simulink model "FieldControl_PID"  (R2022b)
settings: Solver=VariableStepAuto  StartTime=0.0  StopTime=3  MaxStep=1e-5  RelTol=1e-3
model workspace (MAT data in the model file):
  KI_s = 1
  KP_s = 1
undefined symbols (not defined in the file or in its folder): DiscIntNeverNeededParam
libraries: simulink x2, spspowerguiLib x1
settings Model: SimulationMode=accelerator  Creator=AHMED  LastModifiedBy=moham
settings SolverCC: ZeroCrossAlgorithm=Adaptive
settings DebuggingCC: IgnoredZcDiagnostic=none  UnconnectedInputMsg=warning  UnconnectedOutputMsg=warning  UnconnectedLineMsg=warning
settings ModelReferenceCC: EnableRefExpFcnMdlSchedulingChecks=on
settings RTWCC: DLArmComputeVersion=19.05

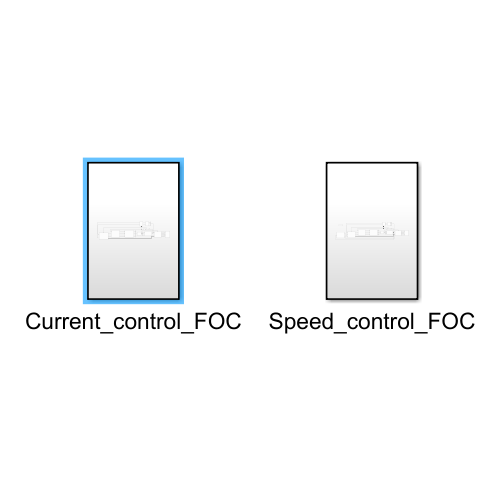
[thumbnail: Simulink's stored preview of the top-level diagram]
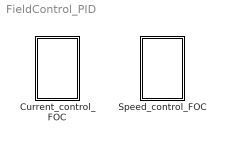
== system FieldControl_PID ==
  Current_control_FOC : Subsystem
  Speed_control_FOC : Subsystem

== system FieldControl_PID/Current_control_FOC ==
  Clark_Transformation : Subsystem
  Control_system : Subsystem
      settings: PortSchema="{\"entries\":[{\"content\":{\"sides\":[{\"content\":{\"connectorIds\":[\"In1\",\"In2\"]},\"type\":\"ConnectorPlacement.EquallySpacedRectSide\",\"uuid\":\"bbdfdf1f-bebb-4c37-9552-0b6c4b897937\"},{\"content\":{\"connectorIds\":[\"Out1\",\"Out2\",\"Out3\"],\"side\":\"RIGHT\"},\"type\":\"ConnectorPlacement.EquallySpacedRectSide\",\"uuid\":\"53bfa961-ba68-4a3a-a1ad-0ed4b4e18017\"},{\"content\":{\"connectorIds\":[\"In3\"],\"side\":\"TOP\"},\"type\":\"ConnectorPlacement.EquallySpacedRectSide\",\"uuid\":\"2095b707-afbd-40f7-b981-0b1948571757\"}]},\"type\":\"ConnectorPlacement.EquallySpacedConnector\",\"uuid\":\"40e57877-c239-4f15-a9c9-ed3794419c45\"}],\"packageUris\":[\"http://schema.mathworks.com/mf0/Connector/R2020b\"],\"version\":\"1.0\"}"
  Demux : Demux  Outputs=3
  Demux1 : Demux  Outputs=3
  Gain : Gain  Gain=2
  Integrator : Integrator
  Inverse_park_clark : Subsystem
  "Inverter " : Subsystem
  Mux : Mux  Inputs=3
  PMSM : Subsystem  mask{Ld=0.0057, Lq=0.0125, lamda_pm=0.123, R=1.2, P=4, J=0.0001, b=0}
  Park_Transformation : Subsystem
      settings: PortSchema="{\"entries\":[{\"content\":{\"sides\":[{\"content\":{\"connectorIds\":[\"In1\",\"In2\"]},\"type\":\"ConnectorPlacement.EquallySpacedRectSide\",\"uuid\":\"a5303260-9056-4ba9-bf21-9d9e68c76aad\"},{\"content\":{\"connectorIds\":[\"Out1\",\"Out2\"],\"side\":\"RIGHT\"},\"type\":\"ConnectorPlacement.EquallySpacedRectSide\",\"uuid\":\"bf8eba39-f781-4672-b99d-9d1cb4b6396f\"},{\"content\":{\"connectorIds\":[],\"side\":\"TOP\"},\"type\":\"ConnectorPlacement.EquallySpacedRectSide\",\"uuid\":\"4985423e-053d-4914-82fe-b9dd9f427f0d\"},{\"content\":{\"connectorIds\":[\"In3\"],\"side\":\"BOTTOM\"},\"type\":\"ConnectorPlacement.EquallySpacedRectSide\",\"uuid\":\"0752c2be-c5bb-44b3-a6b0-4f5b66c2ccb1\"}]},\"type\":\"ConnectorPlacement.EquallySpacedConnector\",\"uuid\":\"0aeb7acd-9c9e-4bf3-9d65-4f157eb3bd0a\"}],\"packageUris\":[\"http://schema.mathworks.com/mf0/Connector/R2020b\"],\"version\":\"1.0\"}"
  SVM : Subsystem
  Scope : Scope  NumInputPorts=8
  Scope_sys : Subsystem
      settings: PortSchema="{\"entries\":[{\"content\":{\"sides\":[{\"content\":{\"connectorIds\":[\"In1\",\"In2\",\"In3\",\"In4\"]},\"type\":\"ConnectorPlacement.EquallySpacedRectSide\",\"uuid\":\"f5ff00d6-72d0-455a-b8b4-a2b5e0f936c9\"},{\"content\":{\"connectorIds\":[\"Out1\",\"Out2\",\"Out3\",\"Out4\",\"Out5\",\"Out6\",\"Out7\",\"Out8\"],\"side\":\"RIGHT\"},\"type\":\"ConnectorPlacement.EquallySpacedRectSide\",\"uuid\":\"90221681-7e43-47d8-9ea8-4435eb27af9a\"},{\"content\":{\"connectorIds\":[\"In5\"],\"side\":\"TOP\"},\"type\":\"ConnectorPlacement.EquallySpacedRectSide\",\"uuid\":\"62fb04f8-341d-442a-bb15-2a5c062453bf\"}]},\"type\":\"ConnectorPlacement.EquallySpacedConnector\",\"uuid\":\"244d1d3d-d937-49d8-9876-c8777bd7e7cc\"}],\"packageUris\":[\"http://schema.mathworks.com/mf0/Connector/R2020b\"],\"version\":\"1.0\"}"
  wires:
  Inverse_park_clark/3(Vc) -> SVM/3(Vc)
  Gain/1 -> Control_system/3(we), Integrator/1
  "Inverter "/1("Voltage ") -> Scope_sys/5("Voltage "), Demux/1
  Inverse_park_clark/2(Vb) -> SVM/2(Vb)
  Demux/3 -> PMSM/3(Vc)
  Clark_Transformation/1(I_alpha) -> Park_Transformation/1(I_alpha)
  SVM/1(S1) -> Mux/1
  Demux/2 -> PMSM/2(Vb)
  SVM/3(S5) -> Mux/3
  Demux1/1 -> Clark_Transformation/1(Ia)
  Clark_Transformation/2(I_beta) -> Park_Transformation/2(I_beta)
  Inverse_park_clark/1(Va) -> SVM/1(Va)
  Mux/1 -> "Inverter "/1("Switches ")
  SVM/2(S3) -> Mux/2
  Control_system/1(Vq) -> Inverse_park_clark/2(Vq)
  Demux1/3 -> Clark_Transformation/3(Ic)
  Integrator/1 -> Park_Transformation/3(theta), Inverse_park_clark/1(theta)
  Control_system/2(Vd) -> Inverse_park_clark/3(Vd)
  Demux1/2 -> Clark_Transformation/2(Ib)
  Demux/1 -> PMSM/1(Va)
  PMSM/1(Stator_currents_Iabc) -> Demux1/1, Scope_sys/1(Iabc)
  PMSM/2(Rotor_speed_Wm) -> Gain/1, Scope_sys/2(Wm)
  PMSM/3(Te) -> Scope_sys/3(Te)
  Park_Transformation/2(I_q) -> Control_system/1(I_q)  "Iq"
  Park_Transformation/1(I_d) -> Control_system/2(I_d)  "Id"
  Control_system/3(Currents) -> Scope_sys/4(Currents)
  Scope_sys/1(Va) -> Scope/1  "Va"
  Scope_sys/2(Vb) -> Scope/2  "Vb"
  Scope_sys/3(Vc) -> Scope/3  "Vc"
  Scope_sys/4(Ia_Ib_Ic) -> Scope/4  "Ia_Ib_Ic"
  Scope_sys/5(Nm) -> Scope/5  "Nm"
  Scope_sys/6(T_ele) -> Scope/6  "Te"
  Scope_sys/7(Iq) -> Scope/7  "Iq"
  Scope_sys/8("Id ") -> Scope/8  "Id"

== system FieldControl_PID/Speed_control_FOC ==
  Clark_Transformation1 : Subsystem
  Current_Control_system : Subsystem
      settings: PortSchema="{\"entries\":[{\"content\":{\"sides\":[{\"content\":{\"connectorIds\":[\"In1\",\"In2\",\"In3\"]},\"type\":\"ConnectorPlacement.EquallySpacedRectSide\",\"uuid\":\"bbdfdf1f-bebb-4c37-9552-0b6c4b897937\"},{\"content\":{\"connectorIds\":[\"Out1\",\"Out2\",\"Out3\"],\"side\":\"RIGHT\"},\"type\":\"ConnectorPlacement.EquallySpacedRectSide\",\"uuid\":\"53bfa961-ba68-4a3a-a1ad-0ed4b4e18017\"},{\"content\":{\"connectorIds\":[\"In4\"],\"side\":\"TOP\"},\"type\":\"ConnectorPlacement.EquallySpacedRectSide\",\"uuid\":\"2095b707-afbd-40f7-b981-0b1948571757\"}]},\"type\":\"ConnectorPlacement.EquallySpacedConnector\",\"uuid\":\"40e57877-c239-4f15-a9c9-ed3794419c45\"}],\"packageUris\":[\"http://schema.mathworks.com/mf0/Connector/R2020b\"],\"version\":\"1.0\"}"
  Demux2 : Demux  Outputs=3
  Demux3 : Demux  Outputs=3
  Gain1 : Gain  Gain=2
  Integrator1 : Integrator
  Inverse_park_clark1 : Subsystem
  Inverter 1 : Subsystem
  Mux1 : Mux  Inputs=3
  PMSM1 : Subsystem  mask{Ld=0.0057, Lq=0.0125, lamda_pm=0.123, R=1.2, P=4, J=0.0001, b=0, TL=4}
  Park_Transformation1 : Subsystem
      settings: PortSchema="{\"entries\":[{\"content\":{\"sides\":[{\"content\":{\"connectorIds\":[\"In1\",\"In2\"]},\"type\":\"ConnectorPlacement.EquallySpacedRectSide\",\"uuid\":\"a5303260-9056-4ba9-bf21-9d9e68c76aad\"},{\"content\":{\"connectorIds\":[\"Out1\",\"Out2\"],\"side\":\"RIGHT\"},\"type\":\"ConnectorPlacement.EquallySpacedRectSide\",\"uuid\":\"bf8eba39-f781-4672-b99d-9d1cb4b6396f\"},{\"content\":{\"connectorIds\":[],\"side\":\"TOP\"},\"type\":\"ConnectorPlacement.EquallySpacedRectSide\",\"uuid\":\"4985423e-053d-4914-82fe-b9dd9f427f0d\"},{\"content\":{\"connectorIds\":[\"In3\"],\"side\":\"BOTTOM\"},\"type\":\"ConnectorPlacement.EquallySpacedRectSide\",\"uuid\":\"0752c2be-c5bb-44b3-a6b0-4f5b66c2ccb1\"}]},\"type\":\"ConnectorPlacement.EquallySpacedConnector\",\"uuid\":\"0aeb7acd-9c9e-4bf3-9d65-4f157eb3bd0a\"}],\"packageUris\":[\"http://schema.mathworks.com/mf0/Connector/R2020b\"],\"version\":\"1.0\"}"
  SVM : Subsystem
  Scope3 : Scope  NumInputPorts=8
  Scope_sys : Subsystem
      settings: PortSchema="{\"entries\":[{\"content\":{\"sides\":[{\"content\":{\"connectorIds\":[\"In1\",\"In2\",\"In3\",\"In4\",\"In5\"]},\"type\":\"ConnectorPlacement.EquallySpacedRectSide\",\"uuid\":\"f5ff00d6-72d0-455a-b8b4-a2b5e0f936c9\"},{\"content\":{\"connectorIds\":[\"Out1\",\"Out2\",\"Out3\",\"Out4\",\"Out5\",\"Out6\",\"Out7\",\"Out8\"],\"side\":\"RIGHT\"},\"type\":\"ConnectorPlacement.EquallySpacedRectSide\",\"uuid\":\"90221681-7e43-47d8-9ea8-4435eb27af9a\"},{\"content\":{\"connectorIds\":[\"In6\"],\"side\":\"TOP\"},\"type\":\"ConnectorPlacement.EquallySpacedRectSide\",\"uuid\":\"62fb04f8-341d-442a-bb15-2a5c062453bf\"}]},\"type\":\"ConnectorPlacement.EquallySpacedConnector\",\"uuid\":\"244d1d3d-d937-49d8-9876-c8777bd7e7cc\"}],\"packageUris\":[\"http://schema.mathworks.com/mf0/Connector/R2020b\"],\"version\":\"1.0\"}"
  Speed_Control_system : Subsystem
  powergui : spspowerguiLib/powergui  Priority=1  SimulationMode=Continuous  SampleTime=50e-6  frequency=60  Iterations=50  frequencyindice=0  Pbase=100e6  ErrMax=1e-4  UnitsV=kV  UnitsW=MW  buscounter=0  FunctionMessages=off  echomessages=off  EnableUseOfTLC=off  CurrentSourceSwitches=off  DisableSnubberDevices=off  DisableRonSwitches=off  DisableVfSwitches=off  DisplayEquations=off  AutomaticDiscreteSolvers=off  SolverType=Tustin/Backward Euler (TBE)  Interpol=off  ExternalGateDelay=off  methode=off  Ts=100  x0status=blocks  SPID=on  SwTol=0  HookPort=off  NonlinearTolerance=1e-4  nMaxIteration=100  ContinueOnMaxIteration=off  RestoreLinks=warning  ResistiveCurrentMeasurement=off  Frange=[0:2:500]  Ylog=off  Xlog=on  ShowGrid=off  save=off  variable=ZData  structure=0  ZoomFFT=off  StartTime=0.0  cycles=1  DisplayStyle=1  fundamental=60  FreqAxis=off  MaxFrequency=1000  frequencyindicesteady=1  RmsSteady=1  display=off
  wires:
  Current_Control_system/3(Currents) -> Scope_sys/4(Currents)
  Scope_sys/8("Id ") -> Scope3/8  "Id"
  PMSM1/3(Te) -> Scope_sys/3(Te)
  Scope_sys/2(Vb) -> Scope3/2  "Vb"
  Demux3/3 -> Clark_Transformation1/3(Ic)
  Scope_sys/6(T_ele) -> Scope3/6  "Te"
  Scope_sys/3(Vc) -> Scope3/3  "Vc"
  PMSM1/1(Stator_currents_Iabc) -> Demux3/1, Scope_sys/1(Iabc)
  Scope_sys/1(Va) -> Scope3/1  "Va"
  PMSM1/2(Rotor_speed_Wm) -> Gain1/1, Scope_sys/2(Wm), Speed_Control_system/1(Wm)
  Scope_sys/7(Iq) -> Scope3/7  "Iq"
  Scope_sys/4(Ia_Ib_Ic) -> Scope3/4  "Ia_Ib_Ic"
  Mux1/1 -> Inverter 1/1("Switches ")
  Park_Transformation1/2(I_q) -> Current_Control_system/1(I_q)  "Iq"
  Scope_sys/5(Nm) -> Scope3/5  "Nm"
  Demux2/1 -> PMSM1/1(Va)
  Demux2/3 -> PMSM1/3(Vc)
  Demux3/2 -> Clark_Transformation1/2(Ib)
  Integrator1/1 -> Park_Transformation1/3(theta), Inverse_park_clark1/1(theta)
  Current_Control_system/2(Vd) -> Inverse_park_clark1/3(Vd)
  Clark_Transformation1/2(I_beta) -> Park_Transformation1/2(I_beta)
  Clark_Transformation1/1(I_alpha) -> Park_Transformation1/1(I_alpha)
  Inverter 1/1("Voltage ") -> Scope_sys/6("Voltage "), Demux2/1
  Park_Transformation1/1(I_d) -> Current_Control_system/2(I_d)  "Id"
  SVM/1(S1) -> Mux1/1
  Inverse_park_clark1/2(Vb) -> SVM/2(Vb)
  Inverse_park_clark1/1(Va) -> SVM/1(Va)
  Current_Control_system/1(Vq) -> Inverse_park_clark1/2(Vq)
  SVM/2(S2) -> Mux1/2
  Demux2/2 -> PMSM1/2(Vb)
  SVM/3(S3) -> Mux1/3
  Demux3/1 -> Clark_Transformation1/1(Ia)
  Inverse_park_clark1/3(Vc) -> SVM/3(Vc)
  Gain1/1 -> Current_Control_system/4(we), Integrator1/1
  Speed_Control_system/1(Iq_ref) -> Current_Control_system/3(Iq_ref)
  Speed_Control_system/2(Wm_ref) -> Scope_sys/5(Wm_ref)

== system FieldControl_PID/Current_control_FOC/Clark_Transformation ==
  Ia : Inport
  Ib : Inport  Port=2
  Ic : Inport  Port=3
  Add : Sum  Inputs=+++
  Add1 : Sum
  Gain : Gain  Gain=-0.5
  Gain1 : Gain  Gain=-0.5
  Gain2 : Gain  Gain=2/3
  Gain3 : Gain  Gain=sqrt(3)/2
  Gain4 : Gain  Gain=-sqrt(3)/2
  Gain5 : Gain  Gain=2/3
  I_alpha : Outport
  I_beta : Outport  Port=2
  wires:
  Ib/1 -> Gain3/1, Gain/1
  Ic/1 -> Gain4/1, Gain1/1
  Gain/1 -> Add/2
  Gain1/1 -> Add/3
  Ia/1 -> Add/1
  Add/1 -> Gain2/1
  Gain2/1 -> I_alpha/1
  Gain4/1 -> Add1/2
  Gain3/1 -> Add1/1
  Add1/1 -> Gain5/1
  Gain5/1 -> I_beta/1

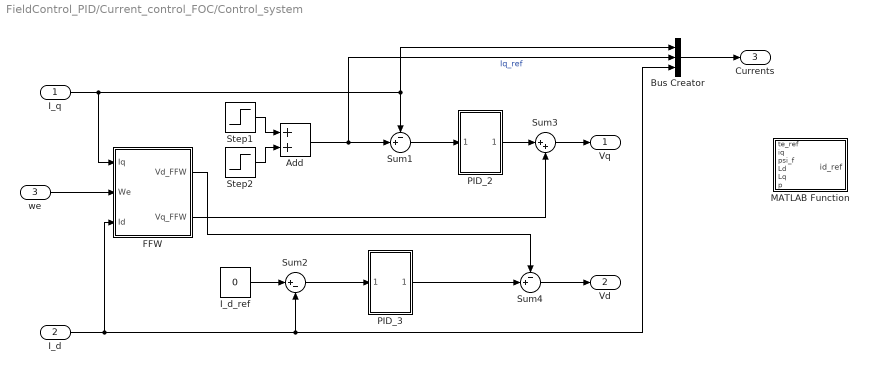
== system FieldControl_PID/Current_control_FOC/Control_system ==
  I_q : Inport
  I_d : Inport  Port=2
  we : Inport  Port=3
  Add : Sum
  Bus Creator : BusCreator  Inputs=3
  FFW : Subsystem
  I_d_ref : Constant  Value=0
  MATLAB Function : MATLAB Function  TreatAsAtomicUnit=on
  PID_2 : Subsystem
  PID_3 : Subsystem
  Step1 : Step  Before=5  After=10  SampleTime=0
  Step2 : Step  Time=2  After=5  SampleTime=0
  Sum1 : Sum  Inputs=-+|
  Sum2 : Sum  Inputs=|+-
  Sum3 : Sum  Inputs=|++
  Sum4 : Sum  Inputs=-+|
  Vq : Outport
  Vd : Outport  Port=2
  Currents : Outport  Port=3
  wires:
  I_q/1 -> FFW/1(Iq), Bus Creator/1, Sum1/1
  Sum1/1 -> PID_2/1(In1)
  I_d/1 -> FFW/3(Id), Bus Creator/3, Sum2/2
  I_d_ref/1 -> Sum2/1
  Sum2/1 -> PID_3/1(In1)
  Add/1 -> Bus Creator/2, Sum1/2  "Iq_ref"
  Bus Creator/1 -> Currents/1
  Sum3/1 -> Vq/1
  PID_3/1(Out1) -> Sum4/2
  Sum4/1 -> Vd/1
  PID_2/1(Out1) -> Sum3/1
  we/1 -> FFW/2(We)
  Step1/1 -> Add/1
  Step2/1 -> Add/2
  FFW/2(Vq_FFW) -> Sum3/2
  FFW/1(Vd_FFW) -> Sum4/1

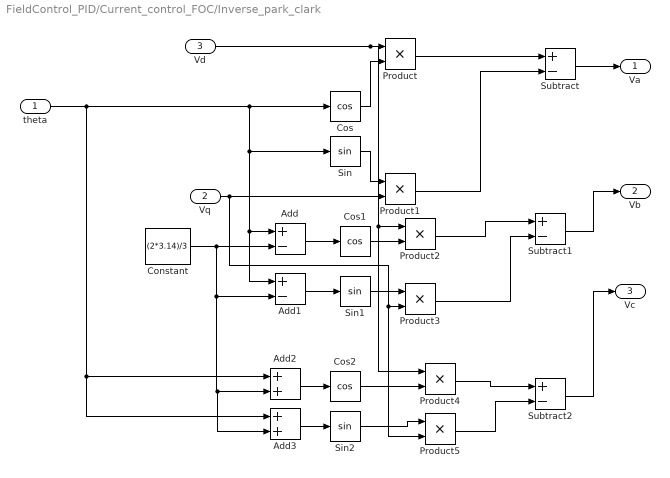
== system FieldControl_PID/Current_control_FOC/Inverse_park_clark ==
  theta : Inport
  Vq : Inport  Port=2
  Vd : Inport  Port=3
  Add : Sum  Inputs=+-
  Add1 : Sum  Inputs=+-
  Add2 : Sum
  Add3 : Sum
  Constant : Constant  Value=(2*3.14)/3
  Cos : Trigonometry  Operator=cos
  Cos1 : Trigonometry  Operator=cos
  Cos2 : Trigonometry  Operator=cos
  Product{,1..5} (6 alike) : Product
  Sin : Trigonometry
  Sin1 : Trigonometry
  Sin2 : Trigonometry
  Subtract : Sum  Inputs=+-
  Subtract1 : Sum  Inputs=+-
  Subtract2 : Sum  Inputs=+-
  Va : Outport
  Vb : Outport  Port=2
  Vc : Outport  Port=3
  wires:
  Subtract/1 -> Va/1
  theta/1 -> Add3/1, Add2/1, Cos/1, Add1/1, Add/1, Sin/1
  Vd/1 -> Product4/1, Product2/1, Product/1
  Cos/1 -> Product/2
  Product/1 -> Subtract/1
  Vq/1 -> Product5/2, Product3/2, Product1/2
  Sin/1 -> Product1/1
  Product1/1 -> Subtract/2
  Add/1 -> Cos1/1
  Add1/1 -> Sin1/1
  Cos1/1 -> Product2/2
  Sin1/1 -> Product3/1
  Product2/1 -> Subtract1/1
  Product3/1 -> Subtract1/2
  Subtract1/1 -> Vb/1
  Constant/1 -> Add3/2, Add2/2, Add1/2, Add/2
  Subtract2/1 -> Vc/1
  Product4/1 -> Subtract2/1
  Product5/1 -> Subtract2/2
  Cos2/1 -> Product4/2
  Sin2/1 -> Product5/1
  Add2/1 -> Cos2/1
  Add3/1 -> Sin2/1

== system FieldControl_PID/Current_control_FOC/Inverter  ==
  "Switches " : Inport
  Fcn : Fcn  Expr=540/3*(2*u(1)-u(2)-u(3))
  Fcn1 : Fcn  Expr=540/3*(2*u(2)-u(1)-u(3))
  Fcn2 : Fcn  Expr=540/3*(2*u(3)-u(2)-u(1))
  Mux1 : Mux  Inputs=3
  "Voltage " : Outport  VectorParamsAs1DForOutWhenUnconnected=off
  wires:
  Mux1/1 -> "Voltage "/1
  Fcn1/1 -> Mux1/2
  "Switches "/1 -> Fcn2/1, Fcn1/1, Fcn/1
  Fcn/1 -> Mux1/1
  Fcn2/1 -> Mux1/3

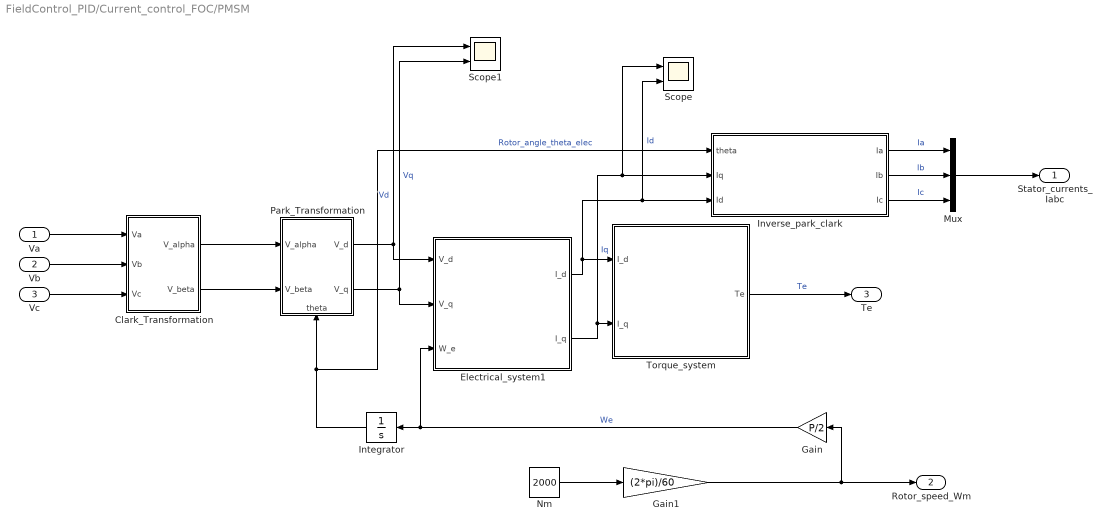
== system FieldControl_PID/Current_control_FOC/PMSM ==
  Va : Inport
  Vb : Inport  Port=2
  Vc : Inport  Port=3
  Clark_Transformation : Subsystem
  Electrical_system1 : Subsystem
  Gain : Gain  Gain=P/2
  Gain1 : Gain  Gain=(2*pi)/60
  Integrator : Integrator
  Inverse_park_clark : Subsystem
  Mux : Mux  Inputs=3
  Nm : Constant  Value=2000
  Park_Transformation : Subsystem
      settings: PortSchema="{\"entries\":[{\"content\":{\"sides\":[{\"content\":{\"connectorIds\":[\"In1\",\"In2\"]},\"type\":\"ConnectorPlacement.EquallySpacedRectSide\",\"uuid\":\"a5303260-9056-4ba9-bf21-9d9e68c76aad\"},{\"content\":{\"connectorIds\":[\"Out1\",\"Out2\"],\"side\":\"RIGHT\"},\"type\":\"ConnectorPlacement.EquallySpacedRectSide\",\"uuid\":\"bf8eba39-f781-4672-b99d-9d1cb4b6396f\"},{\"content\":{\"connectorIds\":[],\"side\":\"TOP\"},\"type\":\"ConnectorPlacement.EquallySpacedRectSide\",\"uuid\":\"4985423e-053d-4914-82fe-b9dd9f427f0d\"},{\"content\":{\"connectorIds\":[\"In3\"],\"side\":\"BOTTOM\"},\"type\":\"ConnectorPlacement.EquallySpacedRectSide\",\"uuid\":\"0752c2be-c5bb-44b3-a6b0-4f5b66c2ccb1\"}]},\"type\":\"ConnectorPlacement.EquallySpacedConnector\",\"uuid\":\"0aeb7acd-9c9e-4bf3-9d65-4f157eb3bd0a\"}],\"packageUris\":[\"http://schema.mathworks.com/mf0/Connector/R2020b\"],\"version\":\"1.0\"}"
  Scope : Scope  NumInputPorts=2
  Scope1 : Scope  NumInputPorts=2
  Torque_system : Subsystem
  Stator_currents_Iabc : Outport
  Rotor_speed_Wm : Outport  Port=2
  Te : Outport  Port=3
  wires:
  Va/1 -> Clark_Transformation/1(Va)
  Vb/1 -> Clark_Transformation/2(Vb)
  Vc/1 -> Clark_Transformation/3(Vc)
  Clark_Transformation/1(V_alpha) -> Park_Transformation/1(V_alpha)
  Clark_Transformation/2(V_beta) -> Park_Transformation/2(V_beta)
  Park_Transformation/1(V_d) -> Electrical_system1/1(V_d), Scope1/1  "Vd"
  Park_Transformation/2(V_q) -> Electrical_system1/2(V_q), Scope1/2  "Vq"
  Electrical_system1/1(I_d) -> Torque_system/1(I_d), Scope/2, Inverse_park_clark/3(Id)  "Id"
  Electrical_system1/2(I_q) -> Scope/1, Inverse_park_clark/2(Iq), Torque_system/2(I_q)  "Iq"
  Torque_system/1(Te) -> Te/1  "Te"
  Gain/1 -> Electrical_system1/3(W_e), Integrator/1  "We"
  Integrator/1 -> Inverse_park_clark/1(theta), Park_Transformation/3(theta)  "Rotor_angle_theta_elec"
  Inverse_park_clark/1(Ia) -> Mux/1  "Ia"
  Inverse_park_clark/2(Ib) -> Mux/2  "Ib"
  Inverse_park_clark/3(Ic) -> Mux/3  "Ic"
  Mux/1 -> Stator_currents_Iabc/1
  Nm/1 -> Gain1/1
  Gain1/1 -> Rotor_speed_Wm/1, Gain/1

== system FieldControl_PID/Current_control_FOC/Park_Transformation ==
  I_alpha : Inport
  I_beta : Inport  Port=2
  theta : Inport  Port=3
  Add : Sum
  Add1 : Sum
  Cos : Trigonometry  Operator=cos
  Cos1 : Trigonometry
  Gain : Gain  Gain=-1
  Product{,1..3} (4 alike) : Product
  I_d : Outport
  I_q : Outport  Port=2
  wires:
  theta/1 -> Cos1/1, Cos/1
  I_alpha/1 -> Product2/1, Product/1
  Cos/1 -> Product3/2, Product/2
  Cos1/1 -> Product2/2, Product1/1
  I_beta/1 -> Product3/1, Product1/2
  Product/1 -> Add/1
  Product1/1 -> Add/2
  Add/1 -> I_d/1
  Product2/1 -> Gain/1
  Gain/1 -> Add1/1
  Product3/1 -> Add1/2
  Add1/1 -> I_q/1

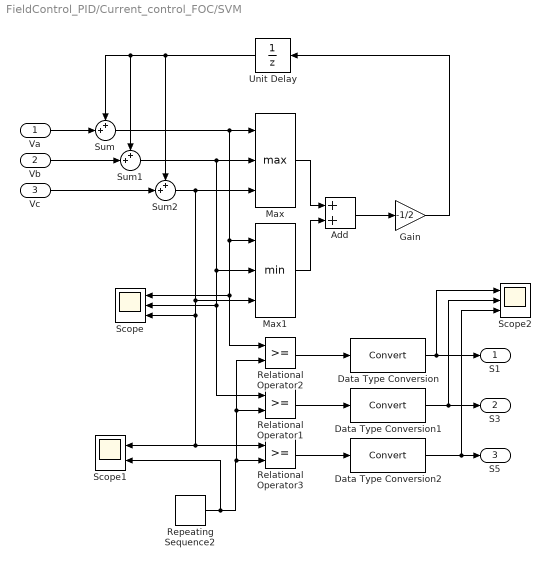
== system FieldControl_PID/Current_control_FOC/SVM ==
  Va : Inport
  Vb : Inport  Port=2
  Vc : Inport  Port=3
  Add : Sum
  Data Type Conversion : DataTypeConversion  SaturateOnIntegerOverflow=off  RndMeth=Floor
  Data Type Conversion1 : DataTypeConversion  SaturateOnIntegerOverflow=off  RndMeth=Floor
  Data Type Conversion2 : DataTypeConversion  SaturateOnIntegerOverflow=off  RndMeth=Floor
  Gain : Gain  Gain=-1/2
  Max : MinMax  Function=max  Inputs=3
  Max1 : MinMax  Inputs=3
  Relational Operator1 : RelationalOperator  OutDataTypeStr=boolean  RndMeth=Simplest  InputSameDT=off
  Relational Operator2 : RelationalOperator  OutDataTypeStr=boolean  RndMeth=Simplest  InputSameDT=off
  Relational Operator3 : RelationalOperator  OutDataTypeStr=boolean  RndMeth=Simplest  InputSameDT=off
  Repeating Sequence2 : simulink/Sources/Repeating Sequence  rep_seq_t=[0 0.5/10000 1/10000]  rep_seq_y=[-280 280 -280]
  Scope : Scope  NumInputPorts=3
  Scope1 : Scope  NumInputPorts=2
  Scope2 : Scope  NumInputPorts=3
  Sum : Sum  Inputs=++|
  Sum1 : Sum  Inputs=++|
  Sum2 : Sum  Inputs=++|
  Unit Delay : UnitDelay  SampleTime=-1  HasFrameUpgradeWarning=on
  S1 : Outport
  S3 : Outport  Port=2
  S5 : Outport  Port=3
  wires:
  Max/1 -> Add/1
  Max1/1 -> Add/2
  Add/1 -> Gain/1
  Data Type Conversion/1 -> Scope2/1, S1/1
  Data Type Conversion1/1 -> Scope2/2, S3/1
  Data Type Conversion2/1 -> Scope2/3, S5/1
  Gain/1 -> Unit Delay/1
  Unit Delay/1 -> Sum1/1, Sum/1, Sum2/1
  Va/1 -> Sum/2
  Vb/1 -> Sum1/2
  Vc/1 -> Sum2/2
  Sum/1 -> Scope/1, Relational Operator2/1, Max1/1, Max/1
  Sum1/1 -> Scope/2, Relational Operator1/1, Max1/2, Max/2
  Sum2/1 -> Scope/3, Scope1/1, Relational Operator3/1, Max1/3, Max/3
  Repeating Sequence2/1 -> Scope1/2, Relational Operator2/2, Relational Operator1/2, Relational Operator3/2
  Relational Operator2/1 -> Data Type Conversion/1
  Relational Operator1/1 -> Data Type Conversion1/1
  Relational Operator3/1 -> Data Type Conversion2/1

== system FieldControl_PID/Current_control_FOC/Scope_sys ==
  Iabc : Inport
  Wm : Inport  Port=2
  Te : Inport  Port=3
  Currents : Inport  Port=4
  "Voltage " : Inport  Port=5
  Bus Selector : BusSelector  OutputSignals=Iq,Iq_ref,Id
  Demux : Demux  Outputs=3
  Gain : Gain  Gain=60/(2*pi)
  Mux : Mux  Inputs=2
  Va : Outport
  Vb : Outport  Port=2
  Vc : Outport  Port=3
  Ia_Ib_Ic : Outport  Port=4
  Nm : Outport  Port=5
  T_ele : Outport  Port=6
  Iq : Outport  Port=7
  "Id " : Outport  Port=8
  wires:
  "Voltage "/1 -> Demux/1
  Demux/1 -> Va/1
  Demux/2 -> Vb/1
  Demux/3 -> Vc/1
  Iabc/1 -> Ia_Ib_Ic/1
  Wm/1 -> Gain/1
  Gain/1 -> Nm/1
  Te/1 -> T_ele/1
  Currents/1 -> Bus Selector/1
  Bus Selector/1 -> Mux/1  "<Iq>"
  Bus Selector/2 -> Mux/2  "<Iq_ref>"
  Bus Selector/3 -> "Id "/1  "<Id>"
  Mux/1 -> Iq/1

== system FieldControl_PID/Speed_control_FOC/Clark_Transformation1 ==
  Ia : Inport
  Ib : Inport  Port=2
  Ic : Inport  Port=3
  Add : Sum  Inputs=+++
  Add1 : Sum
  Gain : Gain  Gain=-0.5
  Gain1 : Gain  Gain=-0.5
  Gain2 : Gain  Gain=2/3
  Gain3 : Gain  Gain=sqrt(3)/2
  Gain4 : Gain  Gain=-sqrt(3)/2
  Gain5 : Gain  Gain=2/3
  I_alpha : Outport
  I_beta : Outport  Port=2
  wires:
  Ib/1 -> Gain3/1, Gain/1
  Ic/1 -> Gain4/1, Gain1/1
  Gain/1 -> Add/2
  Gain1/1 -> Add/3
  Ia/1 -> Add/1
  Add/1 -> Gain2/1
  Gain2/1 -> I_alpha/1
  Gain4/1 -> Add1/2
  Gain3/1 -> Add1/1
  Add1/1 -> Gain5/1
  Gain5/1 -> I_beta/1

== system FieldControl_PID/Speed_control_FOC/Current_Control_system ==
  I_q : Inport
  I_d : Inport  Port=2
  Iq_ref : Inport  Port=3
  we : Inport  Port=4
  Bus Creator : BusCreator  Inputs=3
  I_d_ref : Constant  Value=0
  PID_2 : Subsystem
  PID_3 : Subsystem
  Subsystem : Subsystem
  Sum1 : Sum  Inputs=-+|
  Sum2 : Sum  Inputs=|+-
  Sum3 : Sum  Inputs=|++
  Sum4 : Sum  Inputs=-+|
  Vq : Outport
  Vd : Outport  Port=2
  Currents : Outport  Port=3
  wires:
  I_q/1 -> Subsystem/1(Iq), Bus Creator/1, Sum1/1
  Sum1/1 -> PID_2/1(In1)
  I_d/1 -> Subsystem/3(Id), Bus Creator/3, Sum2/2
  Sum2/1 -> PID_3/1(In1)
  Iq_ref/1 -> Bus Creator/2, Sum1/2  "Iq_ref"
  Bus Creator/1 -> Currents/1
  Sum3/1 -> Vq/1
  PID_3/1(Out1) -> Sum4/2
  Sum4/1 -> Vd/1
  PID_2/1(Out1) -> Sum3/1
  we/1 -> Subsystem/2(We)
  Subsystem/1(Vd_FFW) -> Sum4/1
  Subsystem/2(Vq_FFW) -> Sum3/2
  I_d_ref/1 -> Sum2/1

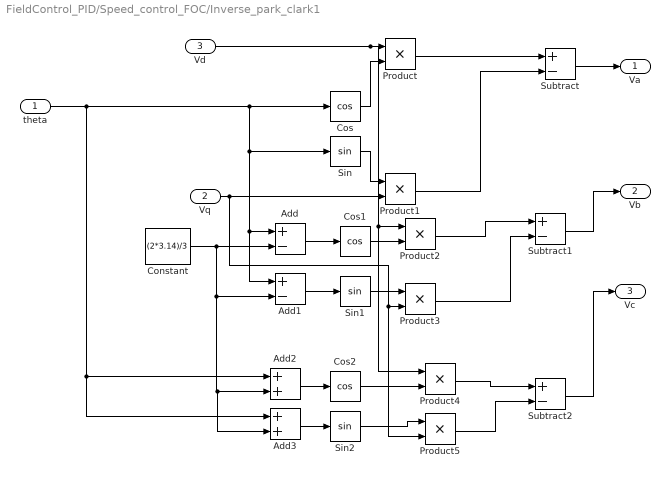
== system FieldControl_PID/Speed_control_FOC/Inverse_park_clark1 ==
  theta : Inport
  Vq : Inport  Port=2
  Vd : Inport  Port=3
  Add : Sum  Inputs=+-
  Add1 : Sum  Inputs=+-
  Add2 : Sum
  Add3 : Sum
  Constant : Constant  Value=(2*3.14)/3
  Cos : Trigonometry  Operator=cos
  Cos1 : Trigonometry  Operator=cos
  Cos2 : Trigonometry  Operator=cos
  Product{,1..5} (6 alike) : Product
  Sin : Trigonometry
  Sin1 : Trigonometry
  Sin2 : Trigonometry
  Subtract : Sum  Inputs=+-
  Subtract1 : Sum  Inputs=+-
  Subtract2 : Sum  Inputs=+-
  Va : Outport
  Vb : Outport  Port=2
  Vc : Outport  Port=3
  wires:
  Subtract/1 -> Va/1
  theta/1 -> Add3/1, Add2/1, Cos/1, Add1/1, Add/1, Sin/1
  Vd/1 -> Product4/1, Product2/1, Product/1
  Cos/1 -> Product/2
  Product/1 -> Subtract/1
  Vq/1 -> Product5/2, Product3/2, Product1/2
  Sin/1 -> Product1/1
  Product1/1 -> Subtract/2
  Add/1 -> Cos1/1
  Add1/1 -> Sin1/1
  Cos1/1 -> Product2/2
  Sin1/1 -> Product3/1
  Product2/1 -> Subtract1/1
  Product3/1 -> Subtract1/2
  Subtract1/1 -> Vb/1
  Constant/1 -> Add3/2, Add2/2, Add1/2, Add/2
  Subtract2/1 -> Vc/1
  Product4/1 -> Subtract2/1
  Product5/1 -> Subtract2/2
  Cos2/1 -> Product4/2
  Sin2/1 -> Product5/1
  Add2/1 -> Cos2/1
  Add3/1 -> Sin2/1

== system FieldControl_PID/Speed_control_FOC/Inverter 1 ==
  "Switches " : Inport
  Fcn : Fcn  Expr=540/3*(2*u(1)-u(2)-u(3))
  Fcn1 : Fcn  Expr=540/3*(2*u(2)-u(1)-u(3))
  Fcn2 : Fcn  Expr=540/3*(2*u(3)-u(2)-u(1))
  Mux1 : Mux  Inputs=3
  "Voltage " : Outport  VectorParamsAs1DForOutWhenUnconnected=off
  wires:
  Mux1/1 -> "Voltage "/1
  Fcn1/1 -> Mux1/2
  "Switches "/1 -> Fcn2/1, Fcn1/1, Fcn/1
  Fcn/1 -> Mux1/1
  Fcn2/1 -> Mux1/3

== system FieldControl_PID/Speed_control_FOC/PMSM1 ==
  Va : Inport
  Vb : Inport  Port=2
  Vc : Inport  Port=3
  Clark_Transformation : Subsystem
  Electrical_system2 : Subsystem
  Gain : Gain  Gain=P/2
  Integrator : Integrator
  Inverse_park_clark : Subsystem
  Mechanical_system : Subsystem
  Mux : Mux  Inputs=3
  Park_Transformation : Subsystem
      settings: PortSchema="{\"entries\":[{\"content\":{\"sides\":[{\"content\":{\"connectorIds\":[\"In1\",\"In2\"]},\"type\":\"ConnectorPlacement.EquallySpacedRectSide\",\"uuid\":\"a5303260-9056-4ba9-bf21-9d9e68c76aad\"},{\"content\":{\"connectorIds\":[\"Out1\",\"Out2\"],\"side\":\"RIGHT\"},\"type\":\"ConnectorPlacement.EquallySpacedRectSide\",\"uuid\":\"bf8eba39-f781-4672-b99d-9d1cb4b6396f\"},{\"content\":{\"connectorIds\":[],\"side\":\"TOP\"},\"type\":\"ConnectorPlacement.EquallySpacedRectSide\",\"uuid\":\"4985423e-053d-4914-82fe-b9dd9f427f0d\"},{\"content\":{\"connectorIds\":[\"In3\"],\"side\":\"BOTTOM\"},\"type\":\"ConnectorPlacement.EquallySpacedRectSide\",\"uuid\":\"0752c2be-c5bb-44b3-a6b0-4f5b66c2ccb1\"}]},\"type\":\"ConnectorPlacement.EquallySpacedConnector\",\"uuid\":\"0aeb7acd-9c9e-4bf3-9d65-4f157eb3bd0a\"}],\"packageUris\":[\"http://schema.mathworks.com/mf0/Connector/R2020b\"],\"version\":\"1.0\"}"
  Scope : Scope  NumInputPorts=2
  Scope1 : Scope  NumInputPorts=2
  Torque_system : Subsystem
  Stator_currents_Iabc : Outport
  Rotor_speed_Wm : Outport  Port=2
  Te : Outport  Port=3
  wires:
  Va/1 -> Clark_Transformation/1(Va)
  Vb/1 -> Clark_Transformation/2(Vb)
  Vc/1 -> Clark_Transformation/3(Vc)
  Clark_Transformation/1(V_alpha) -> Park_Transformation/1(V_alpha)
  Clark_Transformation/2(V_beta) -> Park_Transformation/2(V_beta)
  Park_Transformation/1(V_d) -> Electrical_system2/1(V_d), Scope1/1  "Vd"
  Park_Transformation/2(V_q) -> Electrical_system2/2(V_q), Scope1/2  "Vq"
  Electrical_system2/1(I_d) -> Torque_system/1(I_d), Scope/2, Inverse_park_clark/3(Id)  "Id"
  Electrical_system2/2(I_q) -> Scope/1, Inverse_park_clark/2(Iq), Torque_system/2(I_q)  "Iq"
  Torque_system/1(Te) -> Te/1, Mechanical_system/1(Te)  "Te"
  Mechanical_system/1(Wm) -> Gain/1, Rotor_speed_Wm/1  "Wm"
  Gain/1 -> Electrical_system2/3(W_e), Integrator/1  "We"
  Integrator/1 -> Inverse_park_clark/1(theta), Park_Transformation/3(theta)  "Rotor_angle_theta_elec"
  Inverse_park_clark/1(Ia) -> Mux/1  "Ia"
  Inverse_park_clark/2(Ib) -> Mux/2  "Ib"
  Inverse_park_clark/3(Ic) -> Mux/3  "Ic"
  Mux/1 -> Stator_currents_Iabc/1

== system FieldControl_PID/Speed_control_FOC/Park_Transformation1 ==
  I_alpha : Inport
  I_beta : Inport  Port=2
  theta : Inport  Port=3
  Add : Sum
  Add1 : Sum
  Cos : Trigonometry  Operator=cos
  Cos1 : Trigonometry
  Gain : Gain  Gain=-1
  Product{,1..3} (4 alike) : Product
  I_d : Outport
  I_q : Outport  Port=2
  wires:
  theta/1 -> Cos1/1, Cos/1
  I_alpha/1 -> Product2/1, Product/1
  Cos/1 -> Product3/2, Product/2
  Cos1/1 -> Product2/2, Product1/1
  I_beta/1 -> Product3/1, Product1/2
  Product/1 -> Add/1
  Product1/1 -> Add/2
  Add/1 -> I_d/1
  Product2/1 -> Gain/1
  Gain/1 -> Add1/1
  Product3/1 -> Add1/2
  Add1/1 -> I_q/1

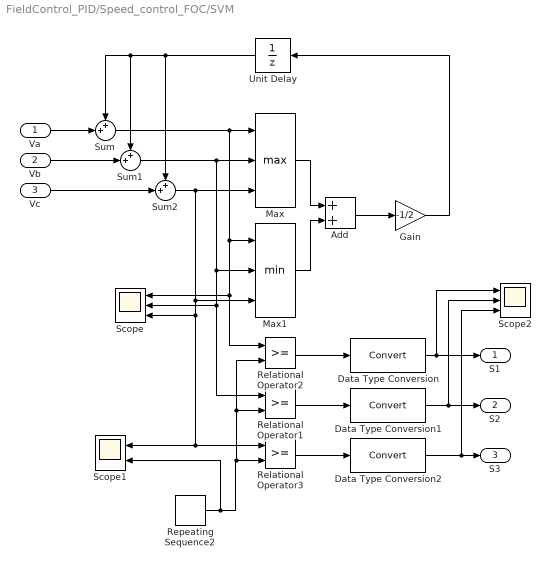
== system FieldControl_PID/Speed_control_FOC/SVM ==
  Va : Inport
  Vb : Inport  Port=2
  Vc : Inport  Port=3
  Add : Sum
  Data Type Conversion : DataTypeConversion  SaturateOnIntegerOverflow=off  RndMeth=Floor
  Data Type Conversion1 : DataTypeConversion  SaturateOnIntegerOverflow=off  RndMeth=Floor
  Data Type Conversion2 : DataTypeConversion  SaturateOnIntegerOverflow=off  RndMeth=Floor
  Gain : Gain  Gain=-1/2
  Max : MinMax  Function=max  Inputs=3
  Max1 : MinMax  Inputs=3
  Relational Operator1 : RelationalOperator  OutDataTypeStr=boolean  RndMeth=Simplest  InputSameDT=off
  Relational Operator2 : RelationalOperator  OutDataTypeStr=boolean  RndMeth=Simplest  InputSameDT=off
  Relational Operator3 : RelationalOperator  OutDataTypeStr=boolean  RndMeth=Simplest  InputSameDT=off
  Repeating Sequence2 : simulink/Sources/Repeating Sequence  rep_seq_t=[0 0.5/10000 1/10000]  rep_seq_y=[-280 280 -280]
  Scope : Scope  NumInputPorts=3
  Scope1 : Scope  NumInputPorts=2
  Scope2 : Scope  NumInputPorts=3
  Sum : Sum  Inputs=++|
  Sum1 : Sum  Inputs=++|
  Sum2 : Sum  Inputs=++|
  Unit Delay : UnitDelay  SampleTime=-1  HasFrameUpgradeWarning=on
  S1 : Outport
  S2 : Outport  Port=2
  S3 : Outport  Port=3
  wires:
  Max/1 -> Add/1
  Max1/1 -> Add/2
  Add/1 -> Gain/1
  Data Type Conversion/1 -> Scope2/1, S1/1
  Data Type Conversion1/1 -> Scope2/2, S2/1
  Data Type Conversion2/1 -> Scope2/3, S3/1
  Gain/1 -> Unit Delay/1
  Unit Delay/1 -> Sum1/1, Sum/1, Sum2/1
  Va/1 -> Sum/2
  Vb/1 -> Sum1/2
  Vc/1 -> Sum2/2
  Sum/1 -> Scope/1, Relational Operator2/1, Max1/1, Max/1
  Sum1/1 -> Scope/2, Relational Operator1/1, Max1/2, Max/2
  Sum2/1 -> Scope/3, Scope1/1, Relational Operator3/1, Max1/3, Max/3
  Repeating Sequence2/1 -> Scope1/2, Relational Operator2/2, Relational Operator1/2, Relational Operator3/2
  Relational Operator2/1 -> Data Type Conversion/1
  Relational Operator1/1 -> Data Type Conversion1/1
  Relational Operator3/1 -> Data Type Conversion2/1

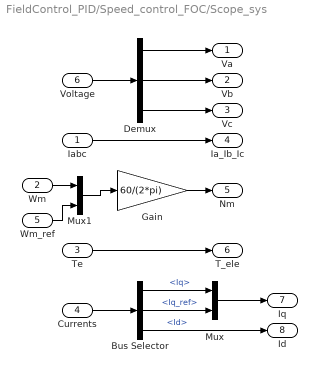
== system FieldControl_PID/Speed_control_FOC/Scope_sys ==
  Iabc : Inport
  Wm : Inport  Port=2
  Te : Inport  Port=3
  Currents : Inport  Port=4
  Wm_ref : Inport  Port=5
  "Voltage " : Inport  Port=6
  Bus Selector : BusSelector  OutputSignals=Iq,Iq_ref,Id
  Demux : Demux  Outputs=3
  Gain : Gain  Gain=60/(2*pi)
  Mux : Mux  Inputs=2
  Mux1 : Mux  Inputs=2
  Va : Outport
  Vb : Outport  Port=2
  Vc : Outport  Port=3
  Ia_Ib_Ic : Outport  Port=4
  Nm : Outport  Port=5
  T_ele : Outport  Port=6
  Iq : Outport  Port=7
  "Id " : Outport  Port=8
  wires:
  "Voltage "/1 -> Demux/1
  Demux/1 -> Va/1
  Demux/2 -> Vb/1
  Demux/3 -> Vc/1
  Iabc/1 -> Ia_Ib_Ic/1
  Gain/1 -> Nm/1
  Te/1 -> T_ele/1
  Currents/1 -> Bus Selector/1
  Bus Selector/1 -> Mux/1  "<Iq>"
  Bus Selector/2 -> Mux/2  "<Iq_ref>"
  Bus Selector/3 -> "Id "/1  "<Id>"
  Mux/1 -> Iq/1
  Wm_ref/1 -> Mux1/2
  Wm/1 -> Mux1/1
  Mux1/1 -> Gain/1

== system FieldControl_PID/Speed_control_FOC/Speed_Control_system ==
  Wm : Inport
  Add : Sum
  PI_system : Subsystem
  Saturation1 : Saturate  UpperLimit=15  LowerLimit=-1
  Step1 : Step  Time=2  After=100  SampleTime=0
  Step2 : Step  Before=200  After=250  SampleTime=0
  Sum : Sum  Inputs=|+-
  Iq_ref : Outport
  Wm_ref : Outport  Port=2
  wires:
  Sum/1 -> PI_system/1(In1)
  Wm/1 -> Sum/2  "Wm"
  Step1/1 -> Add/2
  Add/1 -> Wm_ref/1, Sum/1
  PI_system/1(Iq_ref) -> Saturation1/1
  Saturation1/1 -> Iq_ref/1
  Step2/1 -> Add/1

== system FieldControl_PID/Current_control_FOC/Control_system/FFW ==
  Iq : Inport
  We : Inport  Port=2
  Id : Inport  Port=3
  Add : Sum
  Ld : Gain  Gain=0.0057
  Lq : Gain  Gain=0.0125
  Product : Product
  Product1 : Product
  "delta_pm " : Constant  Value=0.123
  Vd_FFW : Outport
  Vq_FFW : Outport  Port=2
  wires:
  Iq/1 -> Product/1  "Iq"
  We/1 -> Product1/2, Lq/1
  Lq/1 -> Product/2  "We*Lq"
  Product/1 -> Vd_FFW/1
  Product1/1 -> Vq_FFW/1
  Id/1 -> Ld/1
  Ld/1 -> Add/1
  Add/1 -> Product1/1
  "delta_pm "/1 -> Add/2

== system FieldControl_PID/Current_control_FOC/Control_system/PID_2 ==
  In1 : Inport
  Discrete-Time Integrator : DiscreteIntegrator  SampleTime=1/20000  ICPrevOutput=DiscIntNeverNeededParam  ICPrevScaledInput=DiscIntNeverNeededParam
  KI : Gain  Gain=1.2*20000
  Kp : Gain  Gain=0.0125*20000
  Sum : Sum  Inputs=|++
  Out1 : Outport
  wires:
  Sum/1 -> Out1/1
  Discrete-Time Integrator/1 -> Sum/1
  Kp/1 -> Sum/2
  KI/1 -> Discrete-Time Integrator/1
  In1/1 -> KI/1, Kp/1

== system FieldControl_PID/Current_control_FOC/Control_system/PID_3 ==
  In1 : Inport
  Discrete-Time Integrator : DiscreteIntegrator  SampleTime=1/20000  ICPrevOutput=DiscIntNeverNeededParam  ICPrevScaledInput=DiscIntNeverNeededParam
  KI : Gain  Gain=1.2*20000
  Kp : Gain  Gain=0.0057*20000
  Sum : Sum  Inputs=|++
  Out1 : Outport
  wires:
  In1/1 -> Kp/1, KI/1
  KI/1 -> Discrete-Time Integrator/1
  Kp/1 -> Sum/2
  Discrete-Time Integrator/1 -> Sum/1
  Sum/1 -> Out1/1

== system FieldControl_PID/Current_control_FOC/PMSM/Clark_Transformation ==
  Va : Inport
  Vb : Inport  Port=2
  Vc : Inport  Port=3
  Add : Sum  Inputs=+++
  Add1 : Sum
  Gain : Gain  Gain=-0.5
  Gain1 : Gain  Gain=-0.5
  Gain2 : Gain  Gain=2/3
  Gain3 : Gain  Gain=sqrt(3)/2
  Gain4 : Gain  Gain=-sqrt(3)/2
  Gain5 : Gain  Gain=2/3
  V_alpha : Outport
  V_beta : Outport  Port=2
  wires:
  Vb/1 -> Gain3/1, Gain/1
  Vc/1 -> Gain4/1, Gain1/1
  Gain/1 -> Add/2
  Gain1/1 -> Add/3
  Va/1 -> Add/1
  Add/1 -> Gain2/1
  Gain2/1 -> V_alpha/1
  Gain4/1 -> Add1/2
  Gain3/1 -> Add1/1
  Add1/1 -> Gain5/1
  Gain5/1 -> V_beta/1

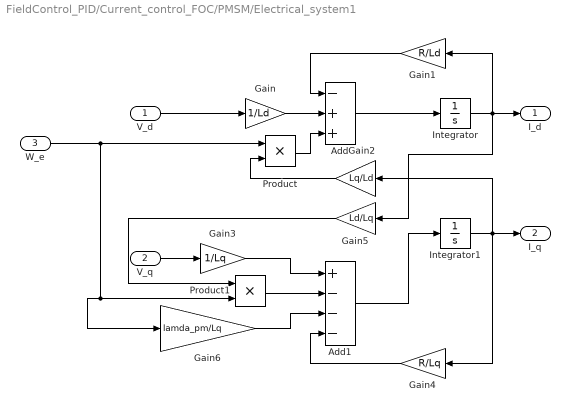
== system FieldControl_PID/Current_control_FOC/PMSM/Electrical_system1 ==
  V_d : Inport
  V_q : Inport  Port=2
  W_e : Inport  Port=3
  Add : Sum  Inputs=-++
  Add1 : Sum  Inputs=+---
  Gain : Gain  Gain=1/Ld
  Gain1 : Gain  Gain=R/Ld
  Gain2 : Gain  Gain=Lq/Ld
  Gain3 : Gain  Gain=1/Lq
  Gain4 : Gain  Gain=R/Lq
  Gain5 : Gain  Gain=Ld/Lq
  Gain6 : Gain  Gain=lamda_pm/Lq
  Integrator : Integrator
  Integrator1 : Integrator
  Product : Product
  Product1 : Product
  I_d : Outport
  I_q : Outport  Port=2
  wires:
  Add1/1 -> Integrator1/1
  Gain6/1 -> Add1/3
  Product1/1 -> Add1/2
  Gain5/1 -> Product1/1
  Gain4/1 -> Add1/4
  Gain3/1 -> Add1/1
  V_q/1 -> Gain3/1
  Product/1 -> Add/3
  W_e/1 -> Product/1, Gain6/1, Product1/2
  Gain2/1 -> Product/2
  Add/1 -> Integrator/1
  Gain1/1 -> Add/1
  Gain/1 -> Add/2
  V_d/1 -> Gain/1
  Integrator1/1 -> I_q/1, Gain2/1, Gain4/1
  Integrator/1 -> I_d/1, Gain1/1, Gain5/1

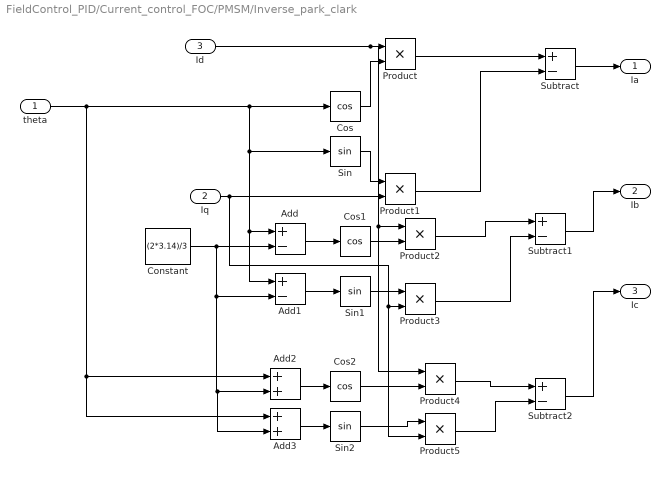
== system FieldControl_PID/Current_control_FOC/PMSM/Inverse_park_clark ==
  theta : Inport
  Iq : Inport  Port=2
  Id : Inport  Port=3
  Add : Sum  Inputs=+-
  Add1 : Sum  Inputs=+-
  Add2 : Sum
  Add3 : Sum
  Constant : Constant  Value=(2*3.14)/3
  Cos : Trigonometry  Operator=cos
  Cos1 : Trigonometry  Operator=cos
  Cos2 : Trigonometry  Operator=cos
  Product{,1..5} (6 alike) : Product
  Sin : Trigonometry
  Sin1 : Trigonometry
  Sin2 : Trigonometry
  Subtract : Sum  Inputs=+-
  Subtract1 : Sum  Inputs=+-
  Subtract2 : Sum  Inputs=+-
  Ia : Outport
  Ib : Outport  Port=2
  Ic : Outport  Port=3
  wires:
  Subtract/1 -> Ia/1
  theta/1 -> Add3/1, Add2/1, Cos/1, Add1/1, Add/1, Sin/1
  Id/1 -> Product4/1, Product2/1, Product/1
  Cos/1 -> Product/2
  Product/1 -> Subtract/1
  Iq/1 -> Product5/2, Product3/2, Product1/2
  Sin/1 -> Product1/1
  Product1/1 -> Subtract/2
  Add/1 -> Cos1/1
  Add1/1 -> Sin1/1
  Cos1/1 -> Product2/2
  Sin1/1 -> Product3/1
  Product2/1 -> Subtract1/1
  Product3/1 -> Subtract1/2
  Subtract1/1 -> Ib/1
  Constant/1 -> Add3/2, Add2/2, Add1/2, Add/2
  Subtract2/1 -> Ic/1
  Product4/1 -> Subtract2/1
  Product5/1 -> Subtract2/2
  Cos2/1 -> Product4/2
  Sin2/1 -> Product5/1
  Add2/1 -> Cos2/1
  Add3/1 -> Sin2/1

== system FieldControl_PID/Current_control_FOC/PMSM/Park_Transformation ==
  V_alpha : Inport
  V_beta : Inport  Port=2
  theta : Inport  Port=3
  Add : Sum
  Add1 : Sum
  Cos : Trigonometry  Operator=cos
  Cos1 : Trigonometry
  Gain : Gain  Gain=-1
  Product{,1..3} (4 alike) : Product
  V_d : Outport
  V_q : Outport  Port=2
  wires:
  theta/1 -> Cos1/1, Cos/1
  V_alpha/1 -> Product2/1, Product/1
  Cos/1 -> Product3/2, Product/2
  Cos1/1 -> Product2/2, Product1/1
  V_beta/1 -> Product3/1, Product1/2
  Product/1 -> Add/1
  Product1/1 -> Add/2
  Add/1 -> V_d/1
  Product2/1 -> Gain/1
  Gain/1 -> Add1/1
  Product3/1 -> Add1/2
  Add1/1 -> V_q/1

== system FieldControl_PID/Current_control_FOC/PMSM/Torque_system ==
  I_d : Inport
  I_q : Inport  Port=2
  Add : Sum  Inputs=+-
  Add1 : Sum
  Constant : Constant  Value=lamda_pm
  Gain : Gain  Gain=(3*P)/4
  Gain1 : Gain  Gain=Ld
  Gain2 : Gain  Gain=Lq
  Product : Product
  Product1 : Product
  Te : Outport
  wires:
  Add/1 -> Gain/1
  Gain/1 -> Te/1
  I_d/1 -> Product1/1, Gain1/1
  Constant/1 -> Add1/2
  Gain1/1 -> Add1/1
  Add1/1 -> Product/2
  I_q/1 -> Gain2/1, Product/1
  Product/1 -> Add/1
  Gain2/1 -> Product1/2
  Product1/1 -> Add/2

== system FieldControl_PID/Speed_control_FOC/Current_Control_system/PID_2 ==
  In1 : Inport
  Discrete-Time Integrator : DiscreteIntegrator  SampleTime=1/20000  ICPrevOutput=DiscIntNeverNeededParam  ICPrevScaledInput=DiscIntNeverNeededParam
  KI : Gain  Gain=1.2*20000
  Kp : Gain  Gain=0.0125*20000
  Sum : Sum  Inputs=|++
  Out1 : Outport
  wires:
  Sum/1 -> Out1/1
  Discrete-Time Integrator/1 -> Sum/1
  Kp/1 -> Sum/2
  KI/1 -> Discrete-Time Integrator/1
  In1/1 -> KI/1, Kp/1

== system FieldControl_PID/Speed_control_FOC/Current_Control_system/PID_3 ==
  In1 : Inport
  Discrete-Time Integrator : DiscreteIntegrator  SampleTime=1/20000  ICPrevOutput=DiscIntNeverNeededParam  ICPrevScaledInput=DiscIntNeverNeededParam
  KI : Gain  Gain=1.2*5000
  Kp : Gain  Gain=0.0057*5000
  Sum : Sum  Inputs=|++
  Out1 : Outport
  wires:
  In1/1 -> Kp/1, KI/1
  KI/1 -> Discrete-Time Integrator/1
  Kp/1 -> Sum/2
  Discrete-Time Integrator/1 -> Sum/1
  Sum/1 -> Out1/1

== system FieldControl_PID/Speed_control_FOC/Current_Control_system/Subsystem ==
  Iq : Inport
  We : Inport  Port=2
  Id : Inport  Port=3
  Add : Sum
  Constant : Constant  Value=0.123
  Gain : Gain  Gain=0.0125
  Gain1 : Gain  Gain=0.0057
  Product : Product
  Product1 : Product
  Vd_FFW : Outport
  Vq_FFW : Outport  Port=2
  wires:
  Iq/1 -> Product/1
  We/1 -> Product1/2, Gain/1
  Gain/1 -> Product/2
  Product/1 -> Vd_FFW/1
  Constant/1 -> Add/2
  Gain1/1 -> Add/1
  Add/1 -> Product1/1
  Product1/1 -> Vq_FFW/1
  Id/1 -> Gain1/1

== system FieldControl_PID/Speed_control_FOC/PMSM1/Clark_Transformation ==
  Va : Inport
  Vb : Inport  Port=2
  Vc : Inport  Port=3
  Add : Sum  Inputs=+++
  Add1 : Sum
  Gain : Gain  Gain=-0.5
  Gain1 : Gain  Gain=-0.5
  Gain2 : Gain  Gain=2/3
  Gain3 : Gain  Gain=sqrt(3)/2
  Gain4 : Gain  Gain=-sqrt(3)/2
  Gain5 : Gain  Gain=2/3
  V_alpha : Outport
  V_beta : Outport  Port=2
  wires:
  Vb/1 -> Gain3/1, Gain/1
  Vc/1 -> Gain4/1, Gain1/1
  Gain/1 -> Add/2
  Gain1/1 -> Add/3
  Va/1 -> Add/1
  Add/1 -> Gain2/1
  Gain2/1 -> V_alpha/1
  Gain4/1 -> Add1/2
  Gain3/1 -> Add1/1
  Add1/1 -> Gain5/1
  Gain5/1 -> V_beta/1

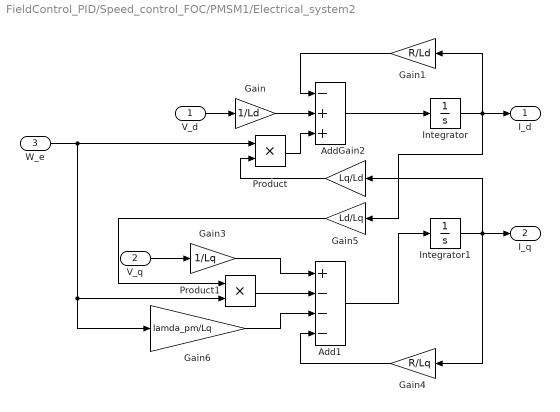
== system FieldControl_PID/Speed_control_FOC/PMSM1/Electrical_system2 ==
  V_d : Inport
  V_q : Inport  Port=2
  W_e : Inport  Port=3
  Add : Sum  Inputs=-++
  Add1 : Sum  Inputs=+---
  Gain : Gain  Gain=1/Ld
  Gain1 : Gain  Gain=R/Ld
  Gain2 : Gain  Gain=Lq/Ld
  Gain3 : Gain  Gain=1/Lq
  Gain4 : Gain  Gain=R/Lq
  Gain5 : Gain  Gain=Ld/Lq
  Gain6 : Gain  Gain=lamda_pm/Lq
  Integrator : Integrator
  Integrator1 : Integrator
  Product : Product
  Product1 : Product
  I_d : Outport
  I_q : Outport  Port=2
  wires:
  Add1/1 -> Integrator1/1
  Gain6/1 -> Add1/3
  Product1/1 -> Add1/2
  Gain5/1 -> Product1/1
  Gain4/1 -> Add1/4
  Gain3/1 -> Add1/1
  V_q/1 -> Gain3/1
  Product/1 -> Add/3
  W_e/1 -> Product/1, Product1/2, Gain6/1
  Gain2/1 -> Product/2
  Add/1 -> Integrator/1
  Gain1/1 -> Add/1
  Gain/1 -> Add/2
  V_d/1 -> Gain/1
  Integrator1/1 -> I_q/1, Gain2/1, Gain4/1
  Integrator/1 -> I_d/1, Gain1/1, Gain5/1

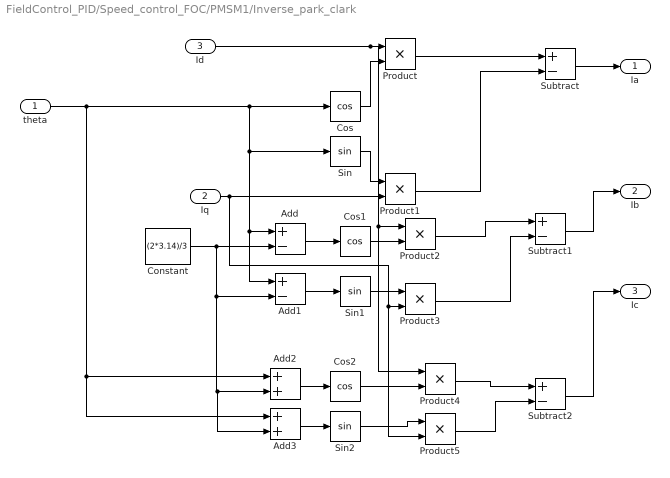
== system FieldControl_PID/Speed_control_FOC/PMSM1/Inverse_park_clark ==
  theta : Inport
  Iq : Inport  Port=2
  Id : Inport  Port=3
  Add : Sum  Inputs=+-
  Add1 : Sum  Inputs=+-
  Add2 : Sum
  Add3 : Sum
  Constant : Constant  Value=(2*3.14)/3
  Cos : Trigonometry  Operator=cos
  Cos1 : Trigonometry  Operator=cos
  Cos2 : Trigonometry  Operator=cos
  Product{,1..5} (6 alike) : Product
  Sin : Trigonometry
  Sin1 : Trigonometry
  Sin2 : Trigonometry
  Subtract : Sum  Inputs=+-
  Subtract1 : Sum  Inputs=+-
  Subtract2 : Sum  Inputs=+-
  Ia : Outport
  Ib : Outport  Port=2
  Ic : Outport  Port=3
  wires:
  Subtract/1 -> Ia/1
  theta/1 -> Add3/1, Add2/1, Cos/1, Add1/1, Add/1, Sin/1
  Id/1 -> Product4/1, Product2/1, Product/1
  Cos/1 -> Product/2
  Product/1 -> Subtract/1
  Iq/1 -> Product5/2, Product3/2, Product1/2
  Sin/1 -> Product1/1
  Product1/1 -> Subtract/2
  Add/1 -> Cos1/1
  Add1/1 -> Sin1/1
  Cos1/1 -> Product2/2
  Sin1/1 -> Product3/1
  Product2/1 -> Subtract1/1
  Product3/1 -> Subtract1/2
  Subtract1/1 -> Ib/1
  Constant/1 -> Add3/2, Add2/2, Add1/2, Add/2
  Subtract2/1 -> Ic/1
  Product4/1 -> Subtract2/1
  Product5/1 -> Subtract2/2
  Cos2/1 -> Product4/2
  Sin2/1 -> Product5/1
  Add2/1 -> Cos2/1
  Add3/1 -> Sin2/1

== system FieldControl_PID/Speed_control_FOC/PMSM1/Mechanical_system ==
  Te : Inport
  Add : Sum  Inputs=+--
  Gain : Gain  Gain=1/J
  Gain1 : Gain  Gain=1/J
  Gain2 : Gain  Gain=b/J
  Integrator : Integrator
  TL : Constant  Value=TL
  Wm : Outport
  wires:
  Integrator/1 -> Wm/1, Gain2/1
  Gain1/1 -> Add/2
  Te/1 -> Gain/1
  TL/1 -> Gain1/1
  Add/1 -> Integrator/1
  Gain/1 -> Add/1
  Gain2/1 -> Add/3

== system FieldControl_PID/Speed_control_FOC/PMSM1/Park_Transformation ==
  V_alpha : Inport
  V_beta : Inport  Port=2
  theta : Inport  Port=3
  Add : Sum
  Add1 : Sum
  Cos : Trigonometry  Operator=cos
  Cos1 : Trigonometry
  Gain : Gain  Gain=-1
  Product{,1..3} (4 alike) : Product
  V_d : Outport
  V_q : Outport  Port=2
  wires:
  theta/1 -> Cos1/1, Cos/1
  V_alpha/1 -> Product2/1, Product/1
  Cos/1 -> Product3/2, Product/2
  Cos1/1 -> Product2/2, Product1/1
  V_beta/1 -> Product3/1, Product1/2
  Product/1 -> Add/1
  Product1/1 -> Add/2
  Add/1 -> V_d/1
  Product2/1 -> Gain/1
  Gain/1 -> Add1/1
  Product3/1 -> Add1/2
  Add1/1 -> V_q/1

== system FieldControl_PID/Speed_control_FOC/PMSM1/Torque_system ==
  I_d : Inport
  I_q : Inport  Port=2
  Add : Sum  Inputs=+-
  Add1 : Sum
  Constant : Constant  Value=lamda_pm
  Gain : Gain  Gain=(3*P)/4
  Gain1 : Gain  Gain=Ld
  Gain2 : Gain  Gain=Lq
  Product : Product
  Product1 : Product
  Te : Outport
  wires:
  Add/1 -> Gain/1
  Gain/1 -> Te/1
  I_d/1 -> Product1/1, Gain1/1
  Constant/1 -> Add1/2
  Gain1/1 -> Add1/1
  Add1/1 -> Product/2
  I_q/1 -> Gain2/1, Product/1
  Product/1 -> Add/1
  Gain2/1 -> Product1/2
  Product1/1 -> Add/2

== system FieldControl_PID/Speed_control_FOC/Speed_Control_system/PI_system ==
  In1 : Inport
  Discrete-Time Integrator : DiscreteIntegrator  SampleTime=1/2000  ICPrevOutput=DiscIntNeverNeededParam  ICPrevScaledInput=DiscIntNeverNeededParam
  KI : Gain  Gain=8
  Kp : Gain  Gain=0.0001*2000*45
  Sum : Sum  Inputs=|++
  Iq_ref : Outport
  wires:
  Sum/1 -> Iq_ref/1
  Discrete-Time Integrator/1 -> Sum/1
  Kp/1 -> Sum/2
  KI/1 -> Discrete-Time Integrator/1
  In1/1 -> KI/1, Kp/1

== matlab function FieldControl_PID/Current_control_FOC/Control_system/MATLAB Function ==
  data: te_ref input; id_ref output; iq input; psi_f input; Ld input; Lq input; p input
function id_ref = mtpa_calculation(te_ref, iq, psi_f, Ld, Lq, p)
    id_ref = -psi_f / (2 * (Ld - Lq)) + sqrt((psi_f / (2 * (Ld - Lq)))^2 + (2 * te_ref) / (3 * p * (Ld - Lq) * iq));
end
